simulink model "modele_qpsk"  (R2024b)
settings: Solver=FixedStepDiscrete  StartTime=0.0  StopTime=(Nsim-1)*Tb  FixedStep=Tpas  RelTol=1e-3
undefined symbols (not defined in the file or in its folder): graine, mappingGray, N0, Tb, Tsym
settings Model: Creator=youka  LastModifiedBy=youka

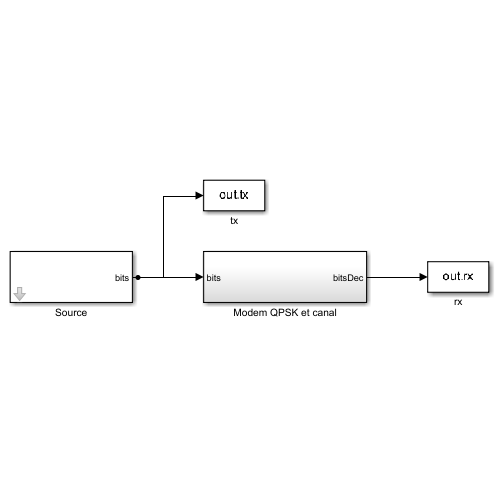
[thumbnail: Simulink's stored preview of the top-level diagram]
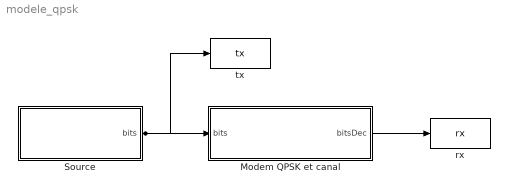
== system modele_qpsk ==
  Modem QPSK et canal : Subsystem
  Source : Subsystem  mask(Source binaire){p_m=0.5, Tb_m=Tb, graine_m=graine}
      mask prompts: p_m "Probabilité d'émettre un 1"; Tb_m "Durée d'un bit Tb (s)"; graine_m "Graine (Seed)"
      mask help: Source binaire sans mémoire : P(1) = p, un bit toutes les Tb secondes.
  rx : ToWorkspace  VariableName=rx  SampleTime=-1
  tx : ToWorkspace  VariableName=tx  SampleTime=-1
  wires:
  Source/1(bits) -> tx/1, Modem QPSK et canal/1(bits)
  Modem QPSK et canal/1(bitsDec) -> rx/1

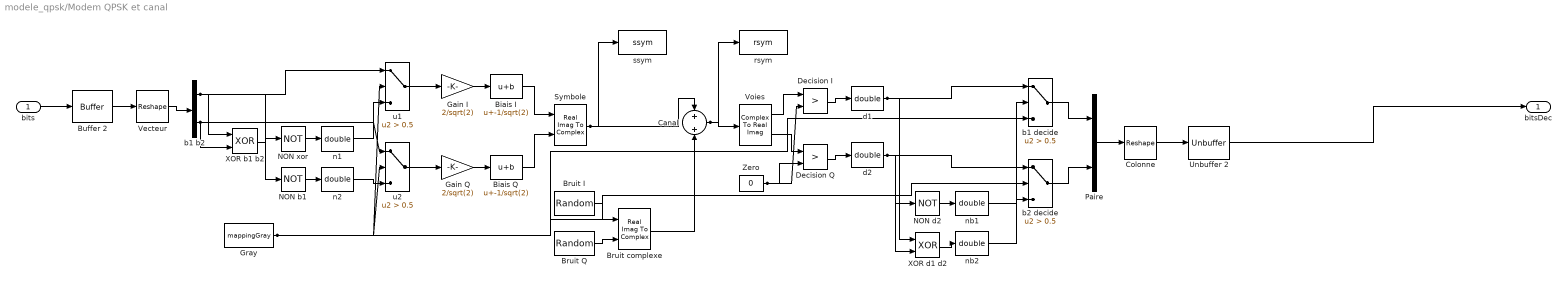
== system modele_qpsk/Modem QPSK et canal ==
  bits : Inport
  Biais I : Bias  Bias=-1/sqrt(2)  SaturateOnIntegerOverflow=off
  Biais Q : Bias  Bias=-1/sqrt(2)  SaturateOnIntegerOverflow=off
  Bruit I : RandomNumber  Variance=N0/2  Seed=graine+1  SampleTime=Tsym
  Bruit Q : RandomNumber  Variance=N0/2  Seed=graine+2  SampleTime=Tsym
  Bruit complexe : RealImagToComplex
  Buffer 2 : Buffer  N=2
  Canal : Sum
  Colonne : Reshape  OutputDimensionality=Column vector (2-D)
  Decision I : RelationalOperator  Operator=>  OutDataTypeStr=boolean  RndMeth=Simplest  InputSameDT=off
  Decision Q : RelationalOperator  Operator=>  OutDataTypeStr=boolean  RndMeth=Simplest  InputSameDT=off
  Gain I : Gain  Gain=2/sqrt(2)
  Gain Q : Gain  Gain=2/sqrt(2)
  Gray : Constant  Value=mappingGray
  NON b1 : Logic  Operator=NOT  AllPortsSameDT=off  OutDataTypeStr=boolean
  NON d2 : Logic  Operator=NOT  AllPortsSameDT=off  OutDataTypeStr=boolean
  NON xor : Logic  Operator=NOT  AllPortsSameDT=off  OutDataTypeStr=boolean
  Paire : Mux  Inputs=2
  Symbole : RealImagToComplex
  Unbuffer 2 : Unbuffer
  Vecteur : Reshape
  Voies : ComplexToRealImag
  XOR b1 b2 : Logic  Operator=XOR  AllPortsSameDT=off  OutDataTypeStr=boolean
  XOR d1 d2 : Logic  Operator=XOR  AllPortsSameDT=off  OutDataTypeStr=boolean
  Zero : Constant  Value=0
  b1 b2 : Demux  Outputs=2
  b1 decide : Switch  Criteria=u2 > Threshold  Threshold=0.5  SaturateOnIntegerOverflow=off  InputSameDT=off
  b2 decide : Switch  Criteria=u2 > Threshold  Threshold=0.5  SaturateOnIntegerOverflow=off  InputSameDT=off
  d1 : DataTypeConversion  OutDataTypeStr=double  SaturateOnIntegerOverflow=off  RndMeth=Floor
  d2 : DataTypeConversion  OutDataTypeStr=double  SaturateOnIntegerOverflow=off  RndMeth=Floor
  n1 : DataTypeConversion  OutDataTypeStr=double  SaturateOnIntegerOverflow=off  RndMeth=Floor
  n2 : DataTypeConversion  OutDataTypeStr=double  SaturateOnIntegerOverflow=off  RndMeth=Floor
  nb1 : DataTypeConversion  OutDataTypeStr=double  SaturateOnIntegerOverflow=off  RndMeth=Floor
  nb2 : DataTypeConversion  OutDataTypeStr=double  SaturateOnIntegerOverflow=off  RndMeth=Floor
  rsym : ToWorkspace  VariableName=rsym  SampleTime=-1
  ssym : ToWorkspace  VariableName=ssym  SampleTime=-1
  u1 : Switch  Criteria=u2 > Threshold  Threshold=0.5  SaturateOnIntegerOverflow=off  InputSameDT=off
  u2 : Switch  Criteria=u2 > Threshold  Threshold=0.5  SaturateOnIntegerOverflow=off  InputSameDT=off
  bitsDec : Outport
  wires:
  bits/1 -> Buffer 2/1
  Buffer 2/1 -> Vecteur/1
  Vecteur/1 -> b1 b2/1
  b1 b2/1 -> XOR b1 b2/1, NON b1/1, u1/1
  b1 b2/2 -> XOR b1 b2/2, u2/1
  XOR b1 b2/1 -> NON xor/1
  NON xor/1 -> n1/1
  NON b1/1 -> n2/1
  Gray/1 -> u1/2, u2/2, b1 decide/2, b2 decide/2
  n1/1 -> u1/3
  n2/1 -> u2/3
  u1/1 -> Gain I/1
  Gain I/1 -> Biais I/1
  Biais I/1 -> Symbole/1
  u2/1 -> Gain Q/1
  Gain Q/1 -> Biais Q/1
  Biais Q/1 -> Symbole/2
  Bruit I/1 -> Bruit complexe/1
  Bruit Q/1 -> Bruit complexe/2
  Symbole/1 -> Canal/1, ssym/1
  Bruit complexe/1 -> Canal/2
  Canal/1 -> rsym/1, Voies/1
  Voies/1 -> Decision I/1
  Zero/1 -> Decision I/2, Decision Q/2
  Voies/2 -> Decision Q/1
  Decision I/1 -> d1/1
  Decision Q/1 -> d2/1
  d2/1 -> NON d2/1, XOR d1 d2/2, b2 decide/1
  NON d2/1 -> nb1/1
  d1/1 -> XOR d1 d2/1, b1 decide/1
  XOR d1 d2/1 -> nb2/1
  nb1/1 -> b1 decide/3
  nb2/1 -> b2 decide/3
  b1 decide/1 -> Paire/1
  b2 decide/1 -> Paire/2
  Paire/1 -> Colonne/1
  Colonne/1 -> Unbuffer 2/1
  Unbuffer 2/1 -> bitsDec/1

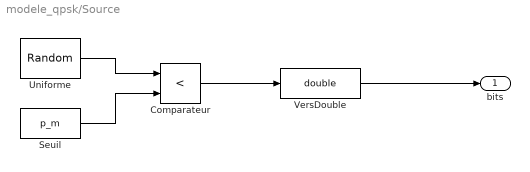
== system modele_qpsk/Source ==
  Comparateur : RelationalOperator  Operator=<  OutDataTypeStr=boolean  RndMeth=Simplest  InputSameDT=off
  Seuil : Constant  Value=p_m  SampleTime=Tb_m
  Uniforme : UniformRandomNumber  Minimum=0  Seed=graine_m  SampleTime=Tb_m
  VersDouble : DataTypeConversion  OutDataTypeStr=double  SaturateOnIntegerOverflow=off  RndMeth=Floor
  bits : Outport
  wires:
  Uniforme/1 -> Comparateur/1
  Seuil/1 -> Comparateur/2
  Comparateur/1 -> VersDouble/1
  VersDouble/1 -> bits/1
